simulink model "Lecture8_example1_sim"  (R2025b)
settings: Solver=VariableStepAuto  StartTime=0.0  StopTime=20  RelTol=1e-3
values from neighbouring files (symbols this model uses):
  C = [1 0 0 0]    [Lecture5_examples.m]    (also in Lecture8_examples.m = [0 1]; Lecture9_examples.m = [0 1]; computationalexampleL02.m = [0 1])
  k = 0    [Lecture10_examples.m]    (also in Lecture6_examples.m = dcgain(H); Lecture8_examples.m = place(A,B,lambda_des); Lecture9_examples.m = place(A,B,lambda_des))
  N = 1/dcgain(sys)    [Lecture8_examples.m]    (also in Lecture9_examples.m = 1/dcgain(sys_c))
libraries: cstblocks x1
settings Model: Creator=WIN10  LastModifiedBy=WIN10

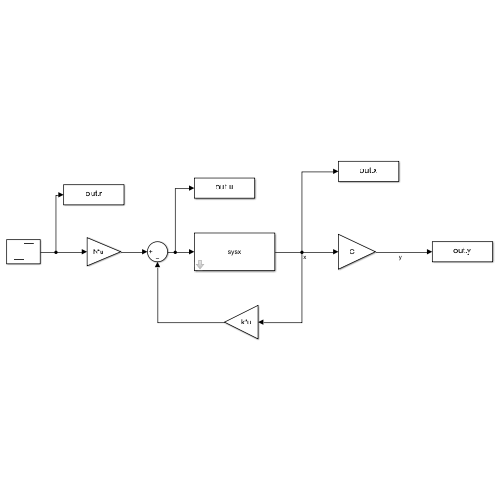
[thumbnail: Simulink's stored preview of the top-level diagram]
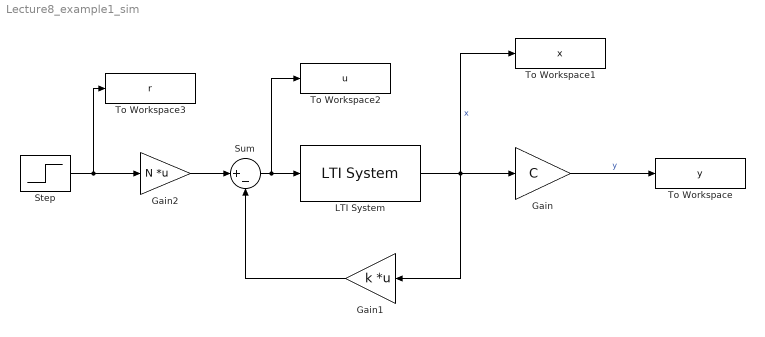
== system Lecture8_example1_sim ==
  Gain : Gain  Gain=C
  Gain1 : Gain  Gain=k  Multiplication=Matrix(K*u)
  Gain2 : Gain  Gain=N  Multiplication=Matrix(K*u)
  LTI System : cstblocks/LTI System  sys=sysx  IC=x0  PadeOrder=0
  Step : Step  Time=0  SampleTime=0
  Sum : Sum  Inputs=|+-
  To Workspace : ToWorkspace  VariableName=y  SaveFormat=Timeseries  SampleTime=-1
  To Workspace1 : ToWorkspace  VariableName=x  SaveFormat=Timeseries  SampleTime=-1
  To Workspace2 : ToWorkspace  VariableName=u  SaveFormat=Timeseries  SampleTime=-1
  To Workspace3 : ToWorkspace  VariableName=r  SaveFormat=Timeseries  SampleTime=-1
  wires:
  LTI System/1 -> Gain1/1, To Workspace1/1, Gain/1  "x"
  Step/1 -> To Workspace3/1, Gain2/1
  Gain2/1 -> Sum/1
  Sum/1 -> To Workspace2/1, LTI System/1
  Gain1/1 -> Sum/2
  Gain/1 -> To Workspace/1  "y"
